simulink model "ASM_Traffic_A11"  (R2026a)
settings: Solver=ode1  StartTime=SIM.tstart.v  StopTime=SIM.tend.v  FixedStep=SIM.StepSize.v
PostLoadFcn:
  | if any(exist('dsrtsu_mdlpostloadfcn', 'file') ~= 0), dsrtsu_mdlpostloadfcn('Execute', bdroot); end
  | try, asm_mdl_postloadfcn(bdroot, 'UpdateModel', 3600); catch, disp(lasterr); end,
InitFcn:
  | , if any(exist('rtifpga_mdlclblib', 'file') ~= 0), rtifpga_mdlclblib('Init', bdroot); end,
  | , if any(exist('dsmpb_private', 'file') ~= 0), dsmpb_private('dsmpb_mdlclblib', 'Init', bdroot); end,
undefined symbols (not defined in the file): _to_, a0b2, ASM_BrakeHydraulics_DemoSystems, ASM_VehicleDynamics_DemoSystems, b98103fe8ad365046cd0, BrakeCircuit, controllerConfig, CPT, Crankshaft, DiscIntNeverNeededParam, dsmsi, FinalDriveAssembly, instance, MDL, ModeSignals, mu, Pos_BrakePedal_Maneuver, rad, RefSignals, s_to_rpm, SIM, SoftECU, Suspension, Tire, Transmission
libraries: ASM_Traffic_lib x135, simulink x98, ASM_Utils_lib x77, ASM_VehicleDynamics_lib x70, ASM_Environment_lib x22, dsmpblib x20, dsmsilib x15, MDLD_Utils_lib x10, ASM_BrakeHydraulics_lib x3, sl_discontinuities x2
(part 46 of 63)

== system ASM_Traffic_A11/Environment/GroundTruth/UserInterface/PAR_Plant/Fellow_Vehicles/Lightstates_Fellow24 ==
  Fellow_Indicator_State[] : Inport
  Brake[] : Constant  Tag=AD:ASM_Sw_SpeedLimit_Source[1Manual|2RoadScenery]  Value=2
  Emergency_Vehicle_Illumination[] : Constant  Tag=AD:ASM_Sw_SpeedLimit_Source[1Manual|2RoadScenery]  Value=2
  Front_Fog_Light[] : Constant  Tag=AD:ASM_Sw_SpeedLimit_Source[1Manual|2RoadScenery]  Value=2
  Head_Light[] : Constant  Tag=AD:ASM_Sw_SpeedLimit_Source[1Manual|2RoadScenery]  Value=2
  High_Beam[] : Constant  Tag=AD:ASM_Sw_SpeedLimit_Source[1Manual|2RoadScenery]  Value=2
  Indicator_State[] : Subsystem
  License_Plate_Illumination_Rear[] : Constant  Tag=AD:ASM_Sw_SpeedLimit_Source[1Manual|2RoadScenery]  Value=2
  Mux : Mux  Inputs=10
  Rear_Fog_Light[] : Constant  Tag=AD:ASM_Sw_SpeedLimit_Source[1Manual|2RoadScenery]  Value=2
  Reversing_Light[] : Constant  Tag=AD:ASM_Sw_SpeedLimit_Source[1Manual|2RoadScenery]  Value=2
  Service_Vehicle_Illumination[] : Constant  Tag=AD:ASM_Sw_SpeedLimit_Source[1Manual|2RoadScenery]  Value=2
  Lightstates[] : Outport  VectorParamsAs1DForOutWhenUnconnected=off
  wires:
  Service_Vehicle_Illumination[]/1 -> Mux/8
  Emergency_Vehicle_Illumination[]/1 -> Mux/7
  License_Plate_Illumination_Rear[]/1 -> Mux/5
  Front_Fog_Light[]/1 -> Mux/3
  Rear_Fog_Light[]/1 -> Mux/6
  Brake[]/1 -> Mux/10
  Head_Light[]/1 -> Mux/4
  High_Beam[]/1 -> Mux/1
  Reversing_Light[]/1 -> Mux/2
  Indicator_State[]/1(Indicator_State[]) -> Mux/9
  Mux/1 -> Lightstates[]/1  "LightStates[]"
  Fellow_Indicator_State[]/1 -> Indicator_State[]/1(Fellow_TurnLights[])

== system ASM_Traffic_A11/Environment/GroundTruth/UserInterface/PAR_Plant/Fellow_Vehicles/Lightstates_Fellow25 ==
  Fellow_Indicator_State[] : Inport
  Brake[] : Constant  Tag=AD:ASM_Sw_SpeedLimit_Source[1Manual|2RoadScenery]  Value=2
  Emergency_Vehicle_Illumination[] : Constant  Tag=AD:ASM_Sw_SpeedLimit_Source[1Manual|2RoadScenery]  Value=2
  Front_Fog_Light[] : Constant  Tag=AD:ASM_Sw_SpeedLimit_Source[1Manual|2RoadScenery]  Value=2
  Head_Light[] : Constant  Tag=AD:ASM_Sw_SpeedLimit_Source[1Manual|2RoadScenery]  Value=2
  High_Beam[] : Constant  Tag=AD:ASM_Sw_SpeedLimit_Source[1Manual|2RoadScenery]  Value=2
  Indicator_State[] : Subsystem
  License_Plate_Illumination_Rear[] : Constant  Tag=AD:ASM_Sw_SpeedLimit_Source[1Manual|2RoadScenery]  Value=2
  Mux : Mux  Inputs=10
  Rear_Fog_Light[] : Constant  Tag=AD:ASM_Sw_SpeedLimit_Source[1Manual|2RoadScenery]  Value=2
  Reversing_Light[] : Constant  Tag=AD:ASM_Sw_SpeedLimit_Source[1Manual|2RoadScenery]  Value=2
  Service_Vehicle_Illumination[] : Constant  Tag=AD:ASM_Sw_SpeedLimit_Source[1Manual|2RoadScenery]  Value=2
  Lightstates[] : Outport  VectorParamsAs1DForOutWhenUnconnected=off
  wires:
  Fellow_Indicator_State[]/1 -> Indicator_State[]/1(Fellow_TurnLights[])
  Mux/1 -> Lightstates[]/1  "LightStates[]"
  Indicator_State[]/1(Indicator_State[]) -> Mux/9
  Reversing_Light[]/1 -> Mux/2
  High_Beam[]/1 -> Mux/1
  Head_Light[]/1 -> Mux/4
  Brake[]/1 -> Mux/10
  Rear_Fog_Light[]/1 -> Mux/6
  Front_Fog_Light[]/1 -> Mux/3
  License_Plate_Illumination_Rear[]/1 -> Mux/5
  Emergency_Vehicle_Illumination[]/1 -> Mux/7
  Service_Vehicle_Illumination[]/1 -> Mux/8

== system ASM_Traffic_A11/Environment/GroundTruth/UserInterface/PAR_Plant/Fellow_Vehicles/Lightstates_Fellow26 ==
  Fellow_Indicator_State[] : Inport
  Brake[] : Constant  Tag=AD:ASM_Sw_SpeedLimit_Source[1Manual|2RoadScenery]  Value=2
  Emergency_Vehicle_Illumination[] : Constant  Tag=AD:ASM_Sw_SpeedLimit_Source[1Manual|2RoadScenery]  Value=2
  Front_Fog_Light[] : Constant  Tag=AD:ASM_Sw_SpeedLimit_Source[1Manual|2RoadScenery]  Value=2
  Head_Light[] : Constant  Tag=AD:ASM_Sw_SpeedLimit_Source[1Manual|2RoadScenery]  Value=2
  High_Beam[] : Constant  Tag=AD:ASM_Sw_SpeedLimit_Source[1Manual|2RoadScenery]  Value=2
  Indicator_State[] : Subsystem
  License_Plate_Illumination_Rear[] : Constant  Tag=AD:ASM_Sw_SpeedLimit_Source[1Manual|2RoadScenery]  Value=2
  Mux : Mux  Inputs=10
  Rear_Fog_Light[] : Constant  Tag=AD:ASM_Sw_SpeedLimit_Source[1Manual|2RoadScenery]  Value=2
  Reversing_Light[] : Constant  Tag=AD:ASM_Sw_SpeedLimit_Source[1Manual|2RoadScenery]  Value=2
  Service_Vehicle_Illumination[] : Constant  Tag=AD:ASM_Sw_SpeedLimit_Source[1Manual|2RoadScenery]  Value=2
  Lightstates[] : Outport  VectorParamsAs1DForOutWhenUnconnected=off
  wires:
  Service_Vehicle_Illumination[]/1 -> Mux/8
  Emergency_Vehicle_Illumination[]/1 -> Mux/7
  License_Plate_Illumination_Rear[]/1 -> Mux/5
  Front_Fog_Light[]/1 -> Mux/3
  Rear_Fog_Light[]/1 -> Mux/6
  Brake[]/1 -> Mux/10
  Head_Light[]/1 -> Mux/4
  High_Beam[]/1 -> Mux/1
  Reversing_Light[]/1 -> Mux/2
  Indicator_State[]/1(Indicator_State[]) -> Mux/9
  Mux/1 -> Lightstates[]/1  "LightStates[]"
  Fellow_Indicator_State[]/1 -> Indicator_State[]/1(Fellow_TurnLights[])

== system ASM_Traffic_A11/Environment/GroundTruth/UserInterface/PAR_Plant/Fellow_Vehicles/Lightstates_Fellow27 ==
  Fellow_Indicator_State[] : Inport
  Brake[] : Constant  Tag=AD:ASM_Sw_SpeedLimit_Source[1Manual|2RoadScenery]  Value=2
  Emergency_Vehicle_Illumination[] : Constant  Tag=AD:ASM_Sw_SpeedLimit_Source[1Manual|2RoadScenery]  Value=2
  Front_Fog_Light[] : Constant  Tag=AD:ASM_Sw_SpeedLimit_Source[1Manual|2RoadScenery]  Value=2
  Head_Light[] : Constant  Tag=AD:ASM_Sw_SpeedLimit_Source[1Manual|2RoadScenery]  Value=2
  High_Beam[] : Constant  Tag=AD:ASM_Sw_SpeedLimit_Source[1Manual|2RoadScenery]  Value=2
  Indicator_State[] : Subsystem
  License_Plate_Illumination_Rear[] : Constant  Tag=AD:ASM_Sw_SpeedLimit_Source[1Manual|2RoadScenery]  Value=2
  Mux : Mux  Inputs=10
  Rear_Fog_Light[] : Constant  Tag=AD:ASM_Sw_SpeedLimit_Source[1Manual|2RoadScenery]  Value=2
  Reversing_Light[] : Constant  Tag=AD:ASM_Sw_SpeedLimit_Source[1Manual|2RoadScenery]  Value=2
  Service_Vehicle_Illumination[] : Constant  Tag=AD:ASM_Sw_SpeedLimit_Source[1Manual|2RoadScenery]  Value=2
  Lightstates[] : Outport  VectorParamsAs1DForOutWhenUnconnected=off
  wires:
  Fellow_Indicator_State[]/1 -> Indicator_State[]/1(Fellow_TurnLights[])
  Mux/1 -> Lightstates[]/1  "LightStates[]"
  Indicator_State[]/1(Indicator_State[]) -> Mux/9
  Reversing_Light[]/1 -> Mux/2
  High_Beam[]/1 -> Mux/1
  Head_Light[]/1 -> Mux/4
  Brake[]/1 -> Mux/10
  Rear_Fog_Light[]/1 -> Mux/6
  Front_Fog_Light[]/1 -> Mux/3
  License_Plate_Illumination_Rear[]/1 -> Mux/5
  Emergency_Vehicle_Illumination[]/1 -> Mux/7
  Service_Vehicle_Illumination[]/1 -> Mux/8

== system ASM_Traffic_A11/Environment/GroundTruth/UserInterface/PAR_Plant/Fellow_Vehicles/Lightstates_Fellow28 ==
  Fellow_Indicator_State[] : Inport
  Brake[] : Constant  Tag=AD:ASM_Sw_SpeedLimit_Source[1Manual|2RoadScenery]  Value=2
  Emergency_Vehicle_Illumination[] : Constant  Tag=AD:ASM_Sw_SpeedLimit_Source[1Manual|2RoadScenery]  Value=2
  Front_Fog_Light[] : Constant  Tag=AD:ASM_Sw_SpeedLimit_Source[1Manual|2RoadScenery]  Value=2
  Head_Light[] : Constant  Tag=AD:ASM_Sw_SpeedLimit_Source[1Manual|2RoadScenery]  Value=2
  High_Beam[] : Constant  Tag=AD:ASM_Sw_SpeedLimit_Source[1Manual|2RoadScenery]  Value=2
  Indicator_State[] : Subsystem
  License_Plate_Illumination_Rear[] : Constant  Tag=AD:ASM_Sw_SpeedLimit_Source[1Manual|2RoadScenery]  Value=2
  Mux : Mux  Inputs=10
  Rear_Fog_Light[] : Constant  Tag=AD:ASM_Sw_SpeedLimit_Source[1Manual|2RoadScenery]  Value=2
  Reversing_Light[] : Constant  Tag=AD:ASM_Sw_SpeedLimit_Source[1Manual|2RoadScenery]  Value=2
  Service_Vehicle_Illumination[] : Constant  Tag=AD:ASM_Sw_SpeedLimit_Source[1Manual|2RoadScenery]  Value=2
  Lightstates[] : Outport  VectorParamsAs1DForOutWhenUnconnected=off
  wires:
  Service_Vehicle_Illumination[]/1 -> Mux/8
  Emergency_Vehicle_Illumination[]/1 -> Mux/7
  License_Plate_Illumination_Rear[]/1 -> Mux/5
  Front_Fog_Light[]/1 -> Mux/3
  Rear_Fog_Light[]/1 -> Mux/6
  Brake[]/1 -> Mux/10
  Head_Light[]/1 -> Mux/4
  High_Beam[]/1 -> Mux/1
  Reversing_Light[]/1 -> Mux/2
  Indicator_State[]/1(Indicator_State[]) -> Mux/9
  Mux/1 -> Lightstates[]/1  "LightStates[]"
  Fellow_Indicator_State[]/1 -> Indicator_State[]/1(Fellow_TurnLights[])

== system ASM_Traffic_A11/Environment/GroundTruth/UserInterface/PAR_Plant/Fellow_Vehicles/Lightstates_Fellow29 ==
  Fellow_Indicator_State[] : Inport
  Brake[] : Constant  Tag=AD:ASM_Sw_SpeedLimit_Source[1Manual|2RoadScenery]  Value=2
  Emergency_Vehicle_Illumination[] : Constant  Tag=AD:ASM_Sw_SpeedLimit_Source[1Manual|2RoadScenery]  Value=2
  Front_Fog_Light[] : Constant  Tag=AD:ASM_Sw_SpeedLimit_Source[1Manual|2RoadScenery]  Value=2
  Head_Light[] : Constant  Tag=AD:ASM_Sw_SpeedLimit_Source[1Manual|2RoadScenery]  Value=2
  High_Beam[] : Constant  Tag=AD:ASM_Sw_SpeedLimit_Source[1Manual|2RoadScenery]  Value=2
  Indicator_State[] : Subsystem
  License_Plate_Illumination_Rear[] : Constant  Tag=AD:ASM_Sw_SpeedLimit_Source[1Manual|2RoadScenery]  Value=2
  Mux : Mux  Inputs=10
  Rear_Fog_Light[] : Constant  Tag=AD:ASM_Sw_SpeedLimit_Source[1Manual|2RoadScenery]  Value=2
  Reversing_Light[] : Constant  Tag=AD:ASM_Sw_SpeedLimit_Source[1Manual|2RoadScenery]  Value=2
  Service_Vehicle_Illumination[] : Constant  Tag=AD:ASM_Sw_SpeedLimit_Source[1Manual|2RoadScenery]  Value=2
  Lightstates[] : Outport  VectorParamsAs1DForOutWhenUnconnected=off
  wires:
  Fellow_Indicator_State[]/1 -> Indicator_State[]/1(Fellow_TurnLights[])
  Mux/1 -> Lightstates[]/1  "LightStates[]"
  Indicator_State[]/1(Indicator_State[]) -> Mux/9
  Reversing_Light[]/1 -> Mux/2
  High_Beam[]/1 -> Mux/1
  Head_Light[]/1 -> Mux/4
  Brake[]/1 -> Mux/10
  Rear_Fog_Light[]/1 -> Mux/6
  Front_Fog_Light[]/1 -> Mux/3
  License_Plate_Illumination_Rear[]/1 -> Mux/5
  Emergency_Vehicle_Illumination[]/1 -> Mux/7
  Service_Vehicle_Illumination[]/1 -> Mux/8

== system ASM_Traffic_A11/Environment/GroundTruth/UserInterface/PAR_Plant/Fellow_Vehicles/Lightstates_Fellow3 ==
  Fellow_Indicator_State[] : Inport
  Brake[] : Constant  Tag=AD:ASM_Sw_SpeedLimit_Source[1Manual|2RoadScenery]  Value=2
  Emergency_Vehicle_Illumination[] : Constant  Tag=AD:ASM_Sw_SpeedLimit_Source[1Manual|2RoadScenery]  Value=2
  Front_Fog_Light[] : Constant  Tag=AD:ASM_Sw_SpeedLimit_Source[1Manual|2RoadScenery]  Value=2
  Head_Light[] : Constant  Tag=AD:ASM_Sw_SpeedLimit_Source[1Manual|2RoadScenery]  Value=2
  High_Beam[] : Constant  Tag=AD:ASM_Sw_SpeedLimit_Source[1Manual|2RoadScenery]  Value=2
  Indicator_State[] : Subsystem
  License_Plate_Illumination_Rear[] : Constant  Tag=AD:ASM_Sw_SpeedLimit_Source[1Manual|2RoadScenery]  Value=2
  Mux : Mux  Inputs=10
  Rear_Fog_Light[] : Constant  Tag=AD:ASM_Sw_SpeedLimit_Source[1Manual|2RoadScenery]  Value=2
  Reversing_Light[] : Constant  Tag=AD:ASM_Sw_SpeedLimit_Source[1Manual|2RoadScenery]  Value=2
  Service_Vehicle_Illumination[] : Constant  Tag=AD:ASM_Sw_SpeedLimit_Source[1Manual|2RoadScenery]  Value=2
  Lightstates[] : Outport  VectorParamsAs1DForOutWhenUnconnected=off
  wires:
  Fellow_Indicator_State[]/1 -> Indicator_State[]/1(Fellow_TurnLights[])
  Mux/1 -> Lightstates[]/1  "LightStates[]"
  Indicator_State[]/1(Indicator_State[]) -> Mux/9
  Reversing_Light[]/1 -> Mux/2
  High_Beam[]/1 -> Mux/1
  Head_Light[]/1 -> Mux/4
  Brake[]/1 -> Mux/10
  Rear_Fog_Light[]/1 -> Mux/6
  Front_Fog_Light[]/1 -> Mux/3
  License_Plate_Illumination_Rear[]/1 -> Mux/5
  Emergency_Vehicle_Illumination[]/1 -> Mux/7
  Service_Vehicle_Illumination[]/1 -> Mux/8

== system ASM_Traffic_A11/Environment/GroundTruth/UserInterface/PAR_Plant/Fellow_Vehicles/Lightstates_Fellow30 ==
  Fellow_Indicator_State[] : Inport
  Brake[] : Constant  Tag=AD:ASM_Sw_SpeedLimit_Source[1Manual|2RoadScenery]  Value=2
  Emergency_Vehicle_Illumination[] : Constant  Tag=AD:ASM_Sw_SpeedLimit_Source[1Manual|2RoadScenery]  Value=2
  Front_Fog_Light[] : Constant  Tag=AD:ASM_Sw_SpeedLimit_Source[1Manual|2RoadScenery]  Value=2
  Head_Light[] : Constant  Tag=AD:ASM_Sw_SpeedLimit_Source[1Manual|2RoadScenery]  Value=2
  High_Beam[] : Constant  Tag=AD:ASM_Sw_SpeedLimit_Source[1Manual|2RoadScenery]  Value=2
  Indicator_State[] : Subsystem
  License_Plate_Illumination_Rear[] : Constant  Tag=AD:ASM_Sw_SpeedLimit_Source[1Manual|2RoadScenery]  Value=2
  Mux : Mux  Inputs=10
  Rear_Fog_Light[] : Constant  Tag=AD:ASM_Sw_SpeedLimit_Source[1Manual|2RoadScenery]  Value=2
  Reversing_Light[] : Constant  Tag=AD:ASM_Sw_SpeedLimit_Source[1Manual|2RoadScenery]  Value=2
  Service_Vehicle_Illumination[] : Constant  Tag=AD:ASM_Sw_SpeedLimit_Source[1Manual|2RoadScenery]  Value=2
  Lightstates[] : Outport  VectorParamsAs1DForOutWhenUnconnected=off
  wires:
  Service_Vehicle_Illumination[]/1 -> Mux/8
  Emergency_Vehicle_Illumination[]/1 -> Mux/7
  License_Plate_Illumination_Rear[]/1 -> Mux/5
  Front_Fog_Light[]/1 -> Mux/3
  Rear_Fog_Light[]/1 -> Mux/6
  Brake[]/1 -> Mux/10
  Head_Light[]/1 -> Mux/4
  High_Beam[]/1 -> Mux/1
  Reversing_Light[]/1 -> Mux/2
  Indicator_State[]/1(Indicator_State[]) -> Mux/9
  Mux/1 -> Lightstates[]/1  "LightStates[]"
  Fellow_Indicator_State[]/1 -> Indicator_State[]/1(Fellow_TurnLights[])

== system ASM_Traffic_A11/Environment/GroundTruth/UserInterface/PAR_Plant/Fellow_Vehicles/Lightstates_Fellow4 ==
  Fellow_Indicator_State[] : Inport
  Brake[] : Constant  Tag=AD:ASM_Sw_SpeedLimit_Source[1Manual|2RoadScenery]  Value=2
  Emergency_Vehicle_Illumination[] : Constant  Tag=AD:ASM_Sw_SpeedLimit_Source[1Manual|2RoadScenery]  Value=2
  Front_Fog_Light[] : Constant  Tag=AD:ASM_Sw_SpeedLimit_Source[1Manual|2RoadScenery]  Value=2
  Head_Light[] : Constant  Tag=AD:ASM_Sw_SpeedLimit_Source[1Manual|2RoadScenery]  Value=2
  High_Beam[] : Constant  Tag=AD:ASM_Sw_SpeedLimit_Source[1Manual|2RoadScenery]  Value=2
  Indicator_State[] : Subsystem
  License_Plate_Illumination_Rear[] : Constant  Tag=AD:ASM_Sw_SpeedLimit_Source[1Manual|2RoadScenery]  Value=2
  Mux : Mux  Inputs=10
  Rear_Fog_Light[] : Constant  Tag=AD:ASM_Sw_SpeedLimit_Source[1Manual|2RoadScenery]  Value=2
  Reversing_Light[] : Constant  Tag=AD:ASM_Sw_SpeedLimit_Source[1Manual|2RoadScenery]  Value=2
  Service_Vehicle_Illumination[] : Constant  Tag=AD:ASM_Sw_SpeedLimit_Source[1Manual|2RoadScenery]  Value=2
  Lightstates[] : Outport  VectorParamsAs1DForOutWhenUnconnected=off
  wires:
  Service_Vehicle_Illumination[]/1 -> Mux/8
  Emergency_Vehicle_Illumination[]/1 -> Mux/7
  License_Plate_Illumination_Rear[]/1 -> Mux/5
  Front_Fog_Light[]/1 -> Mux/3
  Rear_Fog_Light[]/1 -> Mux/6
  Brake[]/1 -> Mux/10
  Head_Light[]/1 -> Mux/4
  High_Beam[]/1 -> Mux/1
  Reversing_Light[]/1 -> Mux/2
  Indicator_State[]/1(Indicator_State[]) -> Mux/9
  Mux/1 -> Lightstates[]/1  "LightStates[]"
  Fellow_Indicator_State[]/1 -> Indicator_State[]/1(Fellow_TurnLights[])

== system ASM_Traffic_A11/Environment/GroundTruth/UserInterface/PAR_Plant/Fellow_Vehicles/Lightstates_Fellow5 ==
  Fellow_Indicator_State[] : Inport
  Brake[] : Constant  Tag=AD:ASM_Sw_SpeedLimit_Source[1Manual|2RoadScenery]  Value=2
  Emergency_Vehicle_Illumination[] : Constant  Tag=AD:ASM_Sw_SpeedLimit_Source[1Manual|2RoadScenery]  Value=2
  Front_Fog_Light[] : Constant  Tag=AD:ASM_Sw_SpeedLimit_Source[1Manual|2RoadScenery]  Value=2
  Head_Light[] : Constant  Tag=AD:ASM_Sw_SpeedLimit_Source[1Manual|2RoadScenery]  Value=2
  High_Beam[] : Constant  Tag=AD:ASM_Sw_SpeedLimit_Source[1Manual|2RoadScenery]  Value=2
  Indicator_State[] : Subsystem
  License_Plate_Illumination_Rear[] : Constant  Tag=AD:ASM_Sw_SpeedLimit_Source[1Manual|2RoadScenery]  Value=2
  Mux : Mux  Inputs=10
  Rear_Fog_Light[] : Constant  Tag=AD:ASM_Sw_SpeedLimit_Source[1Manual|2RoadScenery]  Value=2
  Reversing_Light[] : Constant  Tag=AD:ASM_Sw_SpeedLimit_Source[1Manual|2RoadScenery]  Value=2
  Service_Vehicle_Illumination[] : Constant  Tag=AD:ASM_Sw_SpeedLimit_Source[1Manual|2RoadScenery]  Value=2
  Lightstates[] : Outport  VectorParamsAs1DForOutWhenUnconnected=off
  wires:
  Fellow_Indicator_State[]/1 -> Indicator_State[]/1(Fellow_TurnLights[])
  Mux/1 -> Lightstates[]/1  "LightStates[]"
  Indicator_State[]/1(Indicator_State[]) -> Mux/9
  Reversing_Light[]/1 -> Mux/2
  High_Beam[]/1 -> Mux/1
  Head_Light[]/1 -> Mux/4
  Brake[]/1 -> Mux/10
  Rear_Fog_Light[]/1 -> Mux/6
  Front_Fog_Light[]/1 -> Mux/3
  License_Plate_Illumination_Rear[]/1 -> Mux/5
  Emergency_Vehicle_Illumination[]/1 -> Mux/7
  Service_Vehicle_Illumination[]/1 -> Mux/8

== system ASM_Traffic_A11/Environment/GroundTruth/UserInterface/PAR_Plant/Fellow_Vehicles/Lightstates_Fellow6 ==
  Fellow_Indicator_State[] : Inport
  Brake[] : Constant  Tag=AD:ASM_Sw_SpeedLimit_Source[1Manual|2RoadScenery]  Value=2
  Emergency_Vehicle_Illumination[] : Constant  Tag=AD:ASM_Sw_SpeedLimit_Source[1Manual|2RoadScenery]  Value=2
  Front_Fog_Light[] : Constant  Tag=AD:ASM_Sw_SpeedLimit_Source[1Manual|2RoadScenery]  Value=2
  Head_Light[] : Constant  Tag=AD:ASM_Sw_SpeedLimit_Source[1Manual|2RoadScenery]  Value=2
  High_Beam[] : Constant  Tag=AD:ASM_Sw_SpeedLimit_Source[1Manual|2RoadScenery]  Value=2
  Indicator_State[] : Subsystem
  License_Plate_Illumination_Rear[] : Constant  Tag=AD:ASM_Sw_SpeedLimit_Source[1Manual|2RoadScenery]  Value=2
  Mux : Mux  Inputs=10
  Rear_Fog_Light[] : Constant  Tag=AD:ASM_Sw_SpeedLimit_Source[1Manual|2RoadScenery]  Value=2
  Reversing_Light[] : Constant  Tag=AD:ASM_Sw_SpeedLimit_Source[1Manual|2RoadScenery]  Value=2
  Service_Vehicle_Illumination[] : Constant  Tag=AD:ASM_Sw_SpeedLimit_Source[1Manual|2RoadScenery]  Value=2
  Lightstates[] : Outport  VectorParamsAs1DForOutWhenUnconnected=off
  wires:
  Service_Vehicle_Illumination[]/1 -> Mux/8
  Emergency_Vehicle_Illumination[]/1 -> Mux/7
  License_Plate_Illumination_Rear[]/1 -> Mux/5
  Front_Fog_Light[]/1 -> Mux/3
  Rear_Fog_Light[]/1 -> Mux/6
  Brake[]/1 -> Mux/10
  Head_Light[]/1 -> Mux/4
  High_Beam[]/1 -> Mux/1
  Reversing_Light[]/1 -> Mux/2
  Indicator_State[]/1(Indicator_State[]) -> Mux/9
  Mux/1 -> Lightstates[]/1  "LightStates[]"
  Fellow_Indicator_State[]/1 -> Indicator_State[]/1(Fellow_TurnLights[])

== system ASM_Traffic_A11/Environment/GroundTruth/UserInterface/PAR_Plant/Fellow_Vehicles/Lightstates_Fellow7 ==
  Fellow_Indicator_State[] : Inport
  Brake[] : Constant  Tag=AD:ASM_Sw_SpeedLimit_Source[1Manual|2RoadScenery]  Value=2
  Emergency_Vehicle_Illumination[] : Constant  Tag=AD:ASM_Sw_SpeedLimit_Source[1Manual|2RoadScenery]  Value=2
  Front_Fog_Light[] : Constant  Tag=AD:ASM_Sw_SpeedLimit_Source[1Manual|2RoadScenery]  Value=2
  Head_Light[] : Constant  Tag=AD:ASM_Sw_SpeedLimit_Source[1Manual|2RoadScenery]  Value=2
  High_Beam[] : Constant  Tag=AD:ASM_Sw_SpeedLimit_Source[1Manual|2RoadScenery]  Value=2
  Indicator_State[] : Subsystem
  License_Plate_Illumination_Rear[] : Constant  Tag=AD:ASM_Sw_SpeedLimit_Source[1Manual|2RoadScenery]  Value=2
  Mux : Mux  Inputs=10
  Rear_Fog_Light[] : Constant  Tag=AD:ASM_Sw_SpeedLimit_Source[1Manual|2RoadScenery]  Value=2
  Reversing_Light[] : Constant  Tag=AD:ASM_Sw_SpeedLimit_Source[1Manual|2RoadScenery]  Value=2
  Service_Vehicle_Illumination[] : Constant  Tag=AD:ASM_Sw_SpeedLimit_Source[1Manual|2RoadScenery]  Value=2
  Lightstates[] : Outport  VectorParamsAs1DForOutWhenUnconnected=off
  wires:
  Fellow_Indicator_State[]/1 -> Indicator_State[]/1(Fellow_TurnLights[])
  Mux/1 -> Lightstates[]/1  "LightStates[]"
  Indicator_State[]/1(Indicator_State[]) -> Mux/9
  Reversing_Light[]/1 -> Mux/2
  High_Beam[]/1 -> Mux/1
  Head_Light[]/1 -> Mux/4
  Brake[]/1 -> Mux/10
  Rear_Fog_Light[]/1 -> Mux/6
  Front_Fog_Light[]/1 -> Mux/3
  License_Plate_Illumination_Rear[]/1 -> Mux/5
  Emergency_Vehicle_Illumination[]/1 -> Mux/7
  Service_Vehicle_Illumination[]/1 -> Mux/8

== system ASM_Traffic_A11/Environment/GroundTruth/UserInterface/PAR_Plant/Fellow_Vehicles/Lightstates_Fellow8 ==
  Fellow_Indicator_State[] : Inport
  Brake[] : Constant  Tag=AD:ASM_Sw_SpeedLimit_Source[1Manual|2RoadScenery]  Value=2
  Emergency_Vehicle_Illumination[] : Constant  Tag=AD:ASM_Sw_SpeedLimit_Source[1Manual|2RoadScenery]  Value=2
  Front_Fog_Light[] : Constant  Tag=AD:ASM_Sw_SpeedLimit_Source[1Manual|2RoadScenery]  Value=2
  Head_Light[] : Constant  Tag=AD:ASM_Sw_SpeedLimit_Source[1Manual|2RoadScenery]  Value=2
  High_Beam[] : Constant  Tag=AD:ASM_Sw_SpeedLimit_Source[1Manual|2RoadScenery]  Value=2
  Indicator_State[] : Subsystem
  License_Plate_Illumination_Rear[] : Constant  Tag=AD:ASM_Sw_SpeedLimit_Source[1Manual|2RoadScenery]  Value=2
  Mux : Mux  Inputs=10
  Rear_Fog_Light[] : Constant  Tag=AD:ASM_Sw_SpeedLimit_Source[1Manual|2RoadScenery]  Value=2
  Reversing_Light[] : Constant  Tag=AD:ASM_Sw_SpeedLimit_Source[1Manual|2RoadScenery]  Value=2
  Service_Vehicle_Illumination[] : Constant  Tag=AD:ASM_Sw_SpeedLimit_Source[1Manual|2RoadScenery]  Value=2
  Lightstates[] : Outport  VectorParamsAs1DForOutWhenUnconnected=off
  wires:
  Service_Vehicle_Illumination[]/1 -> Mux/8
  Emergency_Vehicle_Illumination[]/1 -> Mux/7
  License_Plate_Illumination_Rear[]/1 -> Mux/5
  Front_Fog_Light[]/1 -> Mux/3
  Rear_Fog_Light[]/1 -> Mux/6
  Brake[]/1 -> Mux/10
  Head_Light[]/1 -> Mux/4
  High_Beam[]/1 -> Mux/1
  Reversing_Light[]/1 -> Mux/2
  Indicator_State[]/1(Indicator_State[]) -> Mux/9
  Mux/1 -> Lightstates[]/1  "LightStates[]"
  Fellow_Indicator_State[]/1 -> Indicator_State[]/1(Fellow_TurnLights[])

== system ASM_Traffic_A11/Environment/GroundTruth/UserInterface/PAR_Plant/Fellow_Vehicles/Lightstates_Fellow9 ==
  Fellow_Indicator_State[] : Inport
  Brake[] : Constant  Tag=AD:ASM_Sw_SpeedLimit_Source[1Manual|2RoadScenery]  Value=2
  Emergency_Vehicle_Illumination[] : Constant  Tag=AD:ASM_Sw_SpeedLimit_Source[1Manual|2RoadScenery]  Value=2
  Front_Fog_Light[] : Constant  Tag=AD:ASM_Sw_SpeedLimit_Source[1Manual|2RoadScenery]  Value=2
  Head_Light[] : Constant  Tag=AD:ASM_Sw_SpeedLimit_Source[1Manual|2RoadScenery]  Value=2
  High_Beam[] : Constant  Tag=AD:ASM_Sw_SpeedLimit_Source[1Manual|2RoadScenery]  Value=2
  Indicator_State[] : Subsystem
  License_Plate_Illumination_Rear[] : Constant  Tag=AD:ASM_Sw_SpeedLimit_Source[1Manual|2RoadScenery]  Value=2
  Mux : Mux  Inputs=10
  Rear_Fog_Light[] : Constant  Tag=AD:ASM_Sw_SpeedLimit_Source[1Manual|2RoadScenery]  Value=2
  Reversing_Light[] : Constant  Tag=AD:ASM_Sw_SpeedLimit_Source[1Manual|2RoadScenery]  Value=2
  Service_Vehicle_Illumination[] : Constant  Tag=AD:ASM_Sw_SpeedLimit_Source[1Manual|2RoadScenery]  Value=2
  Lightstates[] : Outport  VectorParamsAs1DForOutWhenUnconnected=off
  wires:
  Fellow_Indicator_State[]/1 -> Indicator_State[]/1(Fellow_TurnLights[])
  Mux/1 -> Lightstates[]/1  "LightStates[]"
  Indicator_State[]/1(Indicator_State[]) -> Mux/9
  Reversing_Light[]/1 -> Mux/2
  High_Beam[]/1 -> Mux/1
  Head_Light[]/1 -> Mux/4
  Brake[]/1 -> Mux/10
  Rear_Fog_Light[]/1 -> Mux/6
  Front_Fog_Light[]/1 -> Mux/3
  License_Plate_Illumination_Rear[]/1 -> Mux/5
  Emergency_Vehicle_Illumination[]/1 -> Mux/7
  Service_Vehicle_Illumination[]/1 -> Mux/8

== system ASM_Traffic_A11/Environment/GroundTruth/UserInterface/PAR_Plant/HostVehicle_Data_AutomatedDrivingFunction/AutomatedDrivingFunction_1 ==
  Interface_In : Inport
  Bus Creator : BusCreator  Inputs=10
  Bus Selector1 : BusSelector  OutputSignals=Interface_In.ExternalModel.Driver_Override_ACC_Active[0Off|1On],Interface_In.ExternalModel.Driver_Override_ACC_Reason[0NoOverride|1BrakePedal|2AccPedal],Interface_In.ExternalModel.ACC_State[1OFF|2Standby|3ON]
  Custom_Name_Idx[] : Constant  Value=0
  Custom_State_Idx[] : Constant  Value=0
  Key_1_Idx[] : Constant  Value=0
  Key_2_Idx[] : Constant  Value=0
  Mappings : Subsystem
  Name_Idx[] : Constant  Value=10
  Value_1_Idx[] : Constant  Value=0
  Value_2_Idx[] : Constant  Value=0
  AutomatedDrivingFunction_ACC[] : Outport  VectorParamsAs1DForOutWhenUnconnected=off
  wires:
  Bus Selector1/3 -> Mappings/3(ACC_State[1OFF|2Standby|3ON])  "<ACC_State[1OFF|2Standby|3ON]>"
  Interface_In/1 -> Bus Selector1/1
  Custom_Name_Idx[]/1 -> Bus Creator/5  "Custom_Name_Idx[]"
  Name_Idx[]/1 -> Bus Creator/4  "Name_Idx[]"
  Mappings/2(DriverOverride_Reason_Idx[]) -> Bus Creator/2  "Driver_Override_Reason_Idx[]"
  Bus Creator/1 -> AutomatedDrivingFunction_ACC[]/1
  Custom_State_Idx[]/1 -> Bus Creator/6  "Custom_State_Idx[]"
  Bus Selector1/1 -> Mappings/1(Driver_Override_ACC_Active_In[0Off|1On])  "<Driver_Override_ACC_Active[0Off|1On]>"
  Bus Selector1/2 -> Mappings/2(Driver_Override_ACC_Reason[0NoOverride|1BrakePedal|2AccPedal])  "<Driver_Override_ACC_Reason[0NoOverride|1BrakePedal|2AccPedal]>"
  Mappings/3(State_Idx[]) -> Bus Creator/3  "State_Idx[]"
  Key_1_Idx[]/1 -> Bus Creator/7  "Key_1_Idx[]"
  Value_1_Idx[]/1 -> Bus Creator/8  "Value_1_Idx[]"
  Key_2_Idx[]/1 -> Bus Creator/9  "Key_2_Idx[]"
  Value_2_Idx[]/1 -> Bus Creator/10  "Value_2_Idx[]"
  Mappings/1(Driver_Override_ACC_Active[0Off|1On]) -> Bus Creator/1  "Driver_Override_Active[0Off|1On]"

== system ASM_Traffic_A11/Environment/GroundTruth/UserInterface/PAR_Plant/HostVehicle_Data_AutomatedDrivingFunction/AutomatedDrivingFunction_2 ==
  Interface_In : Inport
  Bus Creator : BusCreator  Inputs=10
  Bus Selector1 : BusSelector  OutputSignals=Interface_In.ExternalModel.Driver_Override_ACC_Active[0Off|1On],Interface_In.ExternalModel.Driver_Override_ACC_Reason[0NoOverride|1BrakePedal|2AccPedal],Interface_In.ExternalModel.AEB[0|1]
  Custom_Name_Idx[] : Constant  Value=0
  Custom_State_Idx[] : Constant  Value=0
  Key_1_Idx[] : Constant  Value=0
  Key_2_Idx[] : Constant  Value=0
  Mappings : Subsystem
  Name_Idx[] : Constant  Value=7
  Value_1_Idx[] : Constant  Value=0
  Value_2_Idx[] : Constant  Value=0
  AutomatedDrivingFunction_AEB[] : Outport  VectorParamsAs1DForOutWhenUnconnected=off
  wires:
  Custom_Name_Idx[]/1 -> Bus Creator/5  "Custom_Name_Idx[]"
  Name_Idx[]/1 -> Bus Creator/4  "Name_Idx[]"
  Custom_State_Idx[]/1 -> Bus Creator/6  "Custom_State_Idx[]"
  Bus Creator/1 -> AutomatedDrivingFunction_AEB[]/1
  Interface_In/1 -> Bus Selector1/1
  Bus Selector1/2 -> Mappings/2(Driver_Override_ACC_Reason[0NoOverride|1BrakePedal|2AccPedal])  "<Driver_Override_ACC_Reason[0NoOverride|1BrakePedal|2AccPedal]>"
  Bus Selector1/3 -> Mappings/3(AEB[0|1])  "<AEB[0|1]>"
  Value_2_Idx[]/1 -> Bus Creator/10  "Value_2_Idx[]"
  Key_2_Idx[]/1 -> Bus Creator/9  "Key_2_Idx[]"
  Value_1_Idx[]/1 -> Bus Creator/8  "Value_1_Idx[]"
  Key_1_Idx[]/1 -> Bus Creator/7  "Key_1_Idx[]"
  Bus Selector1/1 -> Mappings/1(Driver_Override_ACC_Active_In[0Off|1On])  "<Driver_Override_ACC_Active[0Off|1On]>"
  Mappings/1(Driver_Override_ACC_Active[0Off|1On]) -> Bus Creator/1  "Driver_Override_Active[0Off|1On]"
  Mappings/2(DriverOverride_Reason_Idx[]) -> Bus Creator/2  "Driver_Override_Reason_Idx[]"
  Mappings/3(State_Idx[]) -> Bus Creator/3  "State_Idx[]"

== system ASM_Traffic_A11/Environment/GroundTruth/UserInterface/PAR_Plant/HostVehicle_Data_AutomatedDrivingFunction/AutomatedDrivingFunction_3 ==
  Interface_In : Inport
  Bus Creator : BusCreator  Inputs=10
  Bus Selector1 : BusSelector  OutputSignals=Interface_In.ExternalModel.Driver_Override_ACC_Active[0Off|1On],Interface_In.ExternalModel.Driver_Override_ACC_Reason[0NoOverride|1BrakePedal|2AccPedal],Interface_In.ExternalModel.FCW[0|1]
  Custom_Name_Idx[] : Constant  Value=0
  Custom_State_Idx[] : Constant  Value=0
  Key_1_Idx[] : Constant  Value=0
  Key_2_Idx[] : Constant  Value=0
  Mappings : Subsystem
  Name_Idx[] : Constant  Value=3
  Value_1_Idx[] : Constant  Value=0
  Value_2_Idx[] : Constant  Value=0
  AutomatedDrivingFunction_FCW[] : Outport  VectorParamsAs1DForOutWhenUnconnected=off
  wires:
  Custom_Name_Idx[]/1 -> Bus Creator/5  "Custom_Name_Idx[]"
  Name_Idx[]/1 -> Bus Creator/4  "Name_Idx[]"
  Custom_State_Idx[]/1 -> Bus Creator/6  "Custom_State_Idx[]"
  Bus Creator/1 -> AutomatedDrivingFunction_FCW[]/1
  Bus Selector1/3 -> Mappings/3(FCW[0|1])  "<FCW[0|1]>"
  Interface_In/1 -> Bus Selector1/1
  Bus Selector1/2 -> Mappings/2(Driver_Override_ACC_Reason[0NoOverride|1BrakePedal|2AccPedal])  "<Driver_Override_ACC_Reason[0NoOverride|1BrakePedal|2AccPedal]>"
  Value_2_Idx[]/1 -> Bus Creator/10  "Value_2_Idx[]"
  Key_2_Idx[]/1 -> Bus Creator/9  "Key_2_Idx[]"
  Value_1_Idx[]/1 -> Bus Creator/8  "Value_1_Idx[]"
  Key_1_Idx[]/1 -> Bus Creator/7  "Key_1_Idx[]"
  Bus Selector1/1 -> Mappings/1(Driver_Override_ACC_Active_In[0Off|1On])  "<Driver_Override_ACC_Active[0Off|1On]>"
  Mappings/1(Driver_Override_ACC_Active[0Off|1On]) -> Bus Creator/1  "Driver_Override_Active[0Off|1On]"
  Mappings/3(State_Idx[]) -> Bus Creator/3  "State_Idx[]"
  Mappings/2(DriverOverride_Reason_Idx[]) -> Bus Creator/2  "Driver_Override_Reason_Idx[]"

== system ASM_Traffic_A11/Environment/GroundTruth/UserInterface/PAR_Plant/HostVehicle_Data_AutomatedDrivingFunction/AutomatedDrivingFunction_4 ==
  Interface_In : Inport
  Bus Creator : BusCreator  Inputs=10
  Custom_Name_Idx[] : Constant  Value=0
  Custom_State_Idx[] : Constant  Value=0
  Driver_Override_Active[0Off|1On] : Constant  Value=0
  Driver_Override_Reason_Idx[] : Constant  Value=0
  Key_1_Idx[] : Constant  Value=0
  Key_2_Idx[] : Constant  Value=0
  Name_Idx[] : Constant  Value=0
  State_Idx[] : Constant  Value=0
  Terminator : Terminator
  Value_1_Idx[] : Constant  Value=0
  Value_2_Idx[] : Constant  Value=0
  AutomatedDrivingFunction_4[] : Outport  VectorParamsAs1DForOutWhenUnconnected=off
  wires:
  Driver_Override_Active[0Off|1On]/1 -> Bus Creator/1  "Driver_Override_Active[0Off|1On]"
  Driver_Override_Reason_Idx[]/1 -> Bus Creator/2  "Driver_Override_Reason_Idx[]"
  Interface_In/1 -> Terminator/1
  Custom_Name_Idx[]/1 -> Bus Creator/5  "Custom_Name_Idx[]"
  Name_Idx[]/1 -> Bus Creator/4  "Name_Idx[]"
  Custom_State_Idx[]/1 -> Bus Creator/6  "Custom_State_Idx[]"
  State_Idx[]/1 -> Bus Creator/3  "State_Idx[]"
  Bus Creator/1 -> AutomatedDrivingFunction_4[]/1
  Value_2_Idx[]/1 -> Bus Creator/10  "Value_2_Idx[]"
  Key_2_Idx[]/1 -> Bus Creator/9  "Key_2_Idx[]"
  Value_1_Idx[]/1 -> Bus Creator/8  "Value_1_Idx[]"
  Key_1_Idx[]/1 -> Bus Creator/7  "Key_1_Idx[]"

== system ASM_Traffic_A11/Environment/GroundTruth/UserInterface/PAR_Plant/TrafficLight_Counter/TrafficLight_Counter_1 ==
  Bus Creator1 : BusCreator  Inputs=4
  Ext_TrafficLight_Counter_1[] : Constant  Value=0
  Multiport Switch : MultiPortSwitch  DataPortOrder=Zero-based contiguous  Inputs=2  zeroidx=on  SaturateOnIntegerOverflow=off  InputSameDT=off
  Rounding Function : Rounding  Operator=round
  Saturation : Saturate  UpperLimit=2  LowerLimit=0
  Stim_TrafficLight_Counter_1[] : Constant  Value=0
  Sw_TrafficLight_Counter_1[0Stim|1Ext] : Constant  Value=0
  TrafficLight_Counter_1[] : Outport  VectorParamsAs1DForOutWhenUnconnected=off
  wires:
  Bus Creator1/1 -> TrafficLight_Counter_1[]/1
  Stim_TrafficLight_Counter_1[]/1 -> Bus Creator1/2, Multiport Switch/2  "Stim_TrafficLight_Counter_1[]"
  Multiport Switch/1 -> Bus Creator1/4  "TrafficLight_Counter_1[]"
  Saturation/1 -> Multiport Switch/1
  Rounding Function/1 -> Saturation/1
  Ext_TrafficLight_Counter_1[]/1 -> Multiport Switch/3, Bus Creator1/3  "Ext_TrafficLight_Counter_1[]"
  Sw_TrafficLight_Counter_1[0Stim|1Ext]/1 -> Bus Creator1/1, Rounding Function/1  "Sw_TrafficLight_Counter_1[0Stim|1Ext]"

== system ASM_Traffic_A11/Environment/GroundTruth/UserInterface/PAR_Plant/TrafficLight_Counter/TrafficLight_Counter_2 ==
  Bus Creator1 : BusCreator  Inputs=4
  Ext_TrafficLight_Counter_2[] : Constant  Value=0
  Multiport Switch : MultiPortSwitch  DataPortOrder=Zero-based contiguous  Inputs=2  zeroidx=on  SaturateOnIntegerOverflow=off  InputSameDT=off
  Rounding Function : Rounding  Operator=round
  Saturation : Saturate  UpperLimit=2  LowerLimit=0
  Stim_TrafficLight_Counter_2[] : Constant  Value=0
  Sw_TrafficLight_Counter_2[0Stim|1Ext] : Constant  Value=0
  TrafficLight_Counter_2[] : Outport  VectorParamsAs1DForOutWhenUnconnected=off
  wires:
  Sw_TrafficLight_Counter_2[0Stim|1Ext]/1 -> Rounding Function/1, Bus Creator1/1  "Sw_TrafficLight_Counter_2[0Stim|1Ext]"
  Ext_TrafficLight_Counter_2[]/1 -> Bus Creator1/3, Multiport Switch/3  "Ext_TrafficLight_Counter_2[]"
  Rounding Function/1 -> Saturation/1
  Saturation/1 -> Multiport Switch/1
  Multiport Switch/1 -> Bus Creator1/4  "TrafficLight_Counter_2[]"
  Stim_TrafficLight_Counter_2[]/1 -> Multiport Switch/2, Bus Creator1/2  "Stim_TrafficLight_Counter_2[]"
  Bus Creator1/1 -> TrafficLight_Counter_2[]/1

== system ASM_Traffic_A11/Environment/GroundTruth/UserInterface/PAR_Plant/TrafficLight_Counter/TrafficLight_Counter_3 ==
  Bus Creator1 : BusCreator  Inputs=4
  Ext_TrafficLight_Counter_3[] : Constant  Value=0
  Multiport Switch : MultiPortSwitch  DataPortOrder=Zero-based contiguous  Inputs=2  zeroidx=on  SaturateOnIntegerOverflow=off  InputSameDT=off
  Rounding Function : Rounding  Operator=round
  Saturation : Saturate  UpperLimit=2  LowerLimit=0
  Stim_TrafficLight_Counter_3[] : Constant  Value=0
  Sw_TrafficLight_Counter_3[0Stim|1Ext] : Constant  Value=0
  TrafficLight_Counter_3[] : Outport  VectorParamsAs1DForOutWhenUnconnected=off
  wires:
  Bus Creator1/1 -> TrafficLight_Counter_3[]/1
  Stim_TrafficLight_Counter_3[]/1 -> Bus Creator1/2, Multiport Switch/2  "Stim_TrafficLight_Counter_3[]"
  Multiport Switch/1 -> Bus Creator1/4  "TrafficLight_Counter_3[]"
  Saturation/1 -> Multiport Switch/1
  Rounding Function/1 -> Saturation/1
  Ext_TrafficLight_Counter_3[]/1 -> Multiport Switch/3, Bus Creator1/3  "Ext_TrafficLight_Counter_3[]"
  Sw_TrafficLight_Counter_3[0Stim|1Ext]/1 -> Bus Creator1/1, Rounding Function/1  "Sw_TrafficLight_Counter_3[0Stim|1Ext]"

== system ASM_Traffic_A11/Environment/GroundTruth/UserInterface/PAR_Plant/TrafficLight_Counter/TrafficLight_Counter_4 ==
  Bus Creator1 : BusCreator  Inputs=4
  Ext_TrafficLight_Counter_4[] : Constant  Value=0
  Multiport Switch : MultiPortSwitch  DataPortOrder=Zero-based contiguous  Inputs=2  zeroidx=on  SaturateOnIntegerOverflow=off  InputSameDT=off
  Rounding Function : Rounding  Operator=round
  Saturation : Saturate  UpperLimit=2  LowerLimit=0
  Stim_TrafficLight_Counter_4[] : Constant  Value=0
  Sw_TrafficLight_Counter_4[0Stim|1Ext] : Constant  Value=0
  TrafficLight_Counter_4[] : Outport  VectorParamsAs1DForOutWhenUnconnected=off
  wires:
  Sw_TrafficLight_Counter_4[0Stim|1Ext]/1 -> Rounding Function/1, Bus Creator1/1  "Sw_TrafficLight_Counter_4[0Stim|1Ext]"
  Ext_TrafficLight_Counter_4[]/1 -> Bus Creator1/3, Multiport Switch/3  "Ext_TrafficLight_Counter_4[]"
  Rounding Function/1 -> Saturation/1
  Saturation/1 -> Multiport Switch/1
  Multiport Switch/1 -> Bus Creator1/4  "TrafficLight_Counter_4[]"
  Stim_TrafficLight_Counter_4[]/1 -> Multiport Switch/2, Bus Creator1/2  "Stim_TrafficLight_Counter_4[]"
  Bus Creator1/1 -> TrafficLight_Counter_4[]/1

== system ASM_Traffic_A11/Environment/Maneuver/PlantModel/ExternalSegmentEnd/Dist_Front_Min/Replace_NoObjectFound1 ==
  In1 : Inport
  Far_away : Constant  Value=1000
  No_Hinderance : Constant  Value=0
  Relational Operator : RelationalOperator  Operator=<=
  Switch : Switch  Threshold=1  SaturateOnIntegerOverflow=off
  Out1 : Outport  VectorParamsAs1DForOutWhenUnconnected=off
  wires:
  No_Hinderance/1 -> Relational Operator/2
  Relational Operator/1 -> Switch/2
  Far_away/1 -> Switch/1
  In1/1 -> Relational Operator/1, Switch/3
  Switch/1 -> Out1/1

== system ASM_Traffic_A11/Environment/Maneuver/PlantModel/ExternalSegmentEnd/Dist_Rear_Min/Replace_NoObjectFound1 ==
  In1 : Inport
  Far_away : Constant  Value=1000
  No_Hinderance : Constant  Value=0
  Relational Operator : RelationalOperator  Operator=<=
  Switch : Switch  Threshold=1  SaturateOnIntegerOverflow=off
  Out1 : Outport  VectorParamsAs1DForOutWhenUnconnected=off
  wires:
  Switch/1 -> Out1/1
  In1/1 -> Switch/3, Relational Operator/1
  Far_away/1 -> Switch/1
  Relational Operator/1 -> Switch/2
  No_Hinderance/1 -> Relational Operator/2

== system ASM_Traffic_A11/Environment/Maneuver/PlantModel/ExternalSegmentEnd/SegmentEndTrigger/Fishhook ==
  RollRate_Threshold[deg|s] : Inport
  RollRate_Vehicle_CoG[deg|s] : Inport  Port=2
  Abs : Abs
  Fcn_1 : Fcn  Expr=(u[1]>=0.0)*(u[2]<0.0)
  Fcn_2 : Fcn  Expr=(u[1]>0.0)
  Memory1 : UnitDelay  SampleTime=-1
  Memory2 : UnitDelay  SampleTime=-1
  Mux : Mux  Inputs=2
  Product : Product  RndMeth=Zero
  Sum : Sum  Inputs=|-+  SaturateOnIntegerOverflow=on
  SegmentEnd_Fishhook : Outport  VectorParamsAs1DForOutWhenUnconnected=off
  wires:
  Memory1/1 -> Mux/1
  Mux/1 -> Fcn_1/1
  Sum/1 -> Memory1/1, Mux/2
  Abs/1 -> Sum/2
  RollRate_Threshold[deg|s]/1 -> Sum/1, Memory2/1
  RollRate_Vehicle_CoG[deg|s]/1 -> Abs/1
  Memory2/1 -> Fcn_2/1
  Fcn_2/1 -> Product/1
  Fcn_1/1 -> Product/2
  Product/1 -> SegmentEnd_Fishhook/1

== system ASM_Traffic_A11/Environment/Maneuver/PlantModel/ExternalSegmentEnd/SegmentEndTrigger/SaturateAndRound ==
  In : Inport
  Max : Inport  Port=2
  Const_zero : Constant  Value=0
  Data Type Conversion : DataTypeConversion  SaturateOnIntegerOverflow=off  RndMeth=Floor
  Log_and : Logic  Inputs=3  AllPortsSameDT=off  OutDataTypeStr=boolean
  Product : Product  RndMeth=Zero
  RelOp1 : RelationalOperator  Operator===  OutDataTypeStr=boolean  InputSameDT=off
  RelOp2 : RelationalOperator  Operator=<=  OutDataTypeStr=boolean  InputSameDT=off
  RelOp3 : RelationalOperator  OutDataTypeStr=boolean  InputSameDT=off
  Round : Rounding  Operator=round
  ExternalSegmentEnd_Mode[] : Outport  VectorParamsAs1DForOutWhenUnconnected=off
  wires:
  In/1 -> Product/1, RelOp2/1, RelOp3/1, RelOp1/2, Round/1
  Round/1 -> RelOp1/1
  RelOp1/1 -> Log_and/1
  Log_and/1 -> Data Type Conversion/1
  Data Type Conversion/1 -> Product/2
  Const_zero/1 -> RelOp3/2
  RelOp3/1 -> Log_and/2
  RelOp2/1 -> Log_and/3
  Product/1 -> ExternalSegmentEnd_Mode[]/1
  Max/1 -> RelOp2/2

== system ASM_Traffic_A11/Environment/Maneuver/UserInterface/PAR_Plant/ManeuverControl/Enable_ManeuverStart ==
  Sw_StartManeuverAtSimStart[0|1] : Inport
  In : Inport  Port=2
  Data Type Conversion : DataTypeConversion  SaturateOnIntegerOverflow=off  RndMeth=Floor
  Logical Operator : Logic  Operator=OR  AllPortsSameDT=off  OutDataTypeStr=boolean
  Product : Product  Inputs=3
  Step : Step  Time=0.005  SampleTime=SIM.StepSize.v
  Step1 : Step  Time=0.02  InitialValue=1  FinalValue=0  SampleTime=SIM.StepSize.v
  Out : Outport  VectorParamsAs1DForOutWhenUnconnected=off
  wires:
  Step/1 -> Product/2
  Sw_StartManeuverAtSimStart[0|1]/1 -> Product/1
  Product/1 -> Logical Operator/2
  Step1/1 -> Product/3
  Logical Operator/1 -> Data Type Conversion/1
  Data Type Conversion/1 -> Out/1
  In/1 -> Logical Operator/1

== system ASM_Traffic_A11/Environment/Maneuver/UserInterface/PAR_Plant/ManeuverSettings/Replace_BrakePedal_Brake ==
  Sw_MasterBrakeCylinder_Mode[1linear|2physical] : Inport
  Pos_BrakePedal_Brake[%]_ : Inport  Port=2
  Pos_BrakePedal_BrakeUntilStop[%]_ : Inport  Port=3
  Pos_BrakePedal_Replace[%] : Inport  Port=4
  Const_physType : Constant  Value=2
  RelOpConst_physType : RelationalOperator  Operator===  OutDataTypeStr=boolean  InputSameDT=off
  Switch : Switch  Criteria=u2 ~= 0  SaturateOnIntegerOverflow=off  InputSameDT=off
  Switch1 : Switch  Criteria=u2 ~= 0  SaturateOnIntegerOverflow=off  InputSameDT=off
  Pos_BrakePedal_Brake[%] : Outport  VectorParamsAs1DForOutWhenUnconnected=off
  Pos_BrakePedal_BrakeUntilStop[%] : Outport  Port=2  VectorParamsAs1DForOutWhenUnconnected=off
  wires:
  Switch/1 -> Pos_BrakePedal_Brake[%]/1
  Const_physType/1 -> RelOpConst_physType/2
  Sw_MasterBrakeCylinder_Mode[1linear|2physical]/1 -> RelOpConst_physType/1
  RelOpConst_physType/1 -> Switch1/2, Switch/2
  Pos_BrakePedal_Replace[%]/1 -> Switch1/1, Switch/1
  Pos_BrakePedal_Brake[%]_/1 -> Switch/3
  Switch1/1 -> Pos_BrakePedal_BrakeUntilStop[%]/1
  Pos_BrakePedal_BrakeUntilStop[%]_/1 -> Switch1/3

== system ASM_Traffic_A11/Environment/Maneuver/UserInterface/PAR_Plant/ManualControl/StarterPermanentOn_Handling ==
  In1 : Inport
      settings: AttributesFormatString=Mode_StartButtonState[1Stim|2SoftECU]
  In2 : Inport  Port=2
      settings: AttributesFormatString=State_StartButton[-1PowerOff|0Acc|1PowerOn|2StarterOn]
  In3 : Inport  Port=3
  PermanentOn : simulink/Logic and Bit Operations/Compare To Constant  relop===  const=1  OutDataTypeStr=boolean
  StarterOn : Constant  Value=2
  Stim : Constant
  Switch : Switch  Criteria=u2 ~= 0  SaturateOnIntegerOverflow=off  InputSameDT=off
  Switch1 : Switch  Criteria=u2 ~= 0  SaturateOnIntegerOverflow=off  InputSameDT=off
  Out1 : Outport  VectorParamsAs1DForOutWhenUnconnected=off
  Out2 : Outport  Port=2  VectorParamsAs1DForOutWhenUnconnected=off
  wires:
  In1/1 -> Switch/3
  In2/1 -> Switch1/3
  In3/1 -> PermanentOn/1
  PermanentOn/1 -> Switch1/2, Switch/2
  Stim/1 -> Switch/1
  Switch/1 -> Out1/1
  StarterOn/1 -> Switch1/1
  Switch1/1 -> Out2/1

== system ASM_Traffic_A11/Environment/Maneuver/UserInterface/PAR_Plant/ManualControl/TestBench_Switch ==
  In1 : Inport
      settings: AttributesFormatString=Sw_Testbench[0Off|1On]
  In2 : Inport  Port=2
      settings: AttributesFormatString=EngOpNum[]
  Constant : Constant  Value=0
  Switch : Switch  Criteria=u2 ~= 0  SaturateOnIntegerOverflow=off  InputSameDT=off
  Out1 : Outport  VectorParamsAs1DForOutWhenUnconnected=off
  wires:
  Switch/1 -> Out1/1
  In2/1 -> Switch/2
  In1/1 -> Switch/1
  Constant/1 -> Switch/3

== system ASM_Traffic_A11/Environment/Road/UserInterface/PAR_Plant/BasicRoad/Subsystem ==
  Pos_CP_CoorSys_E[:][x;y][m] : Inport
  Add : Sum
  Constant : Constant
  Demux : Demux  Outputs=2
  Gain : Gain  Gain=0
  Terminator : Terminator
  Out1 : Outport  VectorParamsAs1DForOutWhenUnconnected=off
  wires:
  Gain/1 -> Add/1
  Demux/2 -> Terminator/1
  Pos_CP_CoorSys_E[:][x;y][m]/1 -> Demux/1
  Demux/1 -> Gain/1
  Add/1 -> Out1/1
  Constant/1 -> Add/2

== system ASM_Traffic_A11/Environment/Road/UserInterface/PAR_Plant/Objects_DataStreams/DataStream_1 ==
  Maneuver_Signals[] : Inport
  Bus Creator1 : BusCreator  Inputs=4
  Bus Selector : BusSelector  OutputSignals=ManeuverState[]
  Compare To Constant : simulink/Logic and Bit Operations/Compare To Constant  relop=>=  const=3.0  OutDataTypeStr=boolean
  Multiport Switch : MultiPortSwitch  DataPortOrder=Zero-based contiguous  Inputs=2  zeroidx=on  SaturateOnIntegerOverflow=off  InputSameDT=off
  Rounding Function : Rounding  Operator=round
  Saturation : Saturate  UpperLimit=1  LowerLimit=0
  Selector : Selector  InputPortWidth=4  IndexOptions=Index vector (port)  Indices=[1 3]  OutputSizes=1
  Stim_DataStream_1[] : Constant  Value=3
  Sw_DataStream_1[0Stim|1Ext] : Constant
  TrafficLight1_Control : Subsystem
  TrafficLightState[1Red|2Yellow|3RedYellow|4Green] : Constant  Value=[1 3 4 2]  VectorParams1D=off
  DataStream_1[] : Outport  VectorParamsAs1DForOutWhenUnconnected=off
  wires:
  Compare To Constant/1 -> TrafficLight1_Control/1(Reset[])
  Bus Selector/1 -> Compare To Constant/1  "<ManeuverState[]>"
  Maneuver_Signals[]/1 -> Bus Selector/1
  TrafficLightState[1Red|2Yellow|3RedYellow|4Green]/1 -> Selector/1
  Stim_DataStream_1[]/1 -> Selector/2
  Bus Creator1/1 -> DataStream_1[]/1
  Selector/1 -> Bus Creator1/2, Multiport Switch/2  "Stim_DataStream_1[]"
  Multiport Switch/1 -> Bus Creator1/4  "DataStream_1[]"
  Saturation/1 -> Multiport Switch/1
  Rounding Function/1 -> Saturation/1
  TrafficLight1_Control/1(TrafficLightState[1|2|3|4]) -> Multiport Switch/3, Bus Creator1/3  "Ext_DataStream_1[]"
  Sw_DataStream_1[0Stim|1Ext]/1 -> Bus Creator1/1, Rounding Function/1  "Sw_DataStream_1[0Stim|1Ext]"

== system ASM_Traffic_A11/Environment/Road/UserInterface/PAR_Plant/Objects_DataStreams/DataStream_2 ==
  Maneuver_Signals[] : Inport
  Bus Creator1 : BusCreator  Inputs=4
  Bus Selector : BusSelector  OutputSignals=ManeuverState[]
  Compare To Constant : simulink/Logic and Bit Operations/Compare To Constant  relop=>=  const=3.0  OutDataTypeStr=boolean
  Multiport Switch : MultiPortSwitch  DataPortOrder=Zero-based contiguous  Inputs=2  zeroidx=on  SaturateOnIntegerOverflow=off  InputSameDT=off
  Rounding Function : Rounding  Operator=round
  Saturation : Saturate  UpperLimit=1  LowerLimit=0
  Selector : Selector  InputPortWidth=4  IndexOptions=Index vector (port)  Indices=[1 3]  OutputSizes=1
  Stim_DataStream_2[] : Constant  Value=3
  Sw_DataStream_2[0Stim|1Ext] : Constant
  TrafficLight2_Control : Subsystem
  TrafficLightState[1Red|2Yellow|3RedYellow|4Green] : Constant  Value=[1 3 4 2]  VectorParams1D=off
  DataStream_2[] : Outport  VectorParamsAs1DForOutWhenUnconnected=off
  wires:
  Sw_DataStream_2[0Stim|1Ext]/1 -> Rounding Function/1, Bus Creator1/1  "Sw_DataStream_2[0Stim|1Ext]"
  TrafficLight2_Control/1(TrafficLightState[1|2|3|4]) -> Bus Creator1/3, Multiport Switch/3  "Ext_DataStream_2[]"
  Rounding Function/1 -> Saturation/1
  Saturation/1 -> Multiport Switch/1
  Multiport Switch/1 -> Bus Creator1/4  "DataStream_2[]"
  Selector/1 -> Multiport Switch/2, Bus Creator1/2  "Stim_DataStream_2[]"
  Bus Creator1/1 -> DataStream_2[]/1
  Stim_DataStream_2[]/1 -> Selector/2
  Maneuver_Signals[]/1 -> Bus Selector/1
  Bus Selector/1 -> Compare To Constant/1  "<ManeuverState[]>"
  Compare To Constant/1 -> TrafficLight2_Control/1(Reset[])
  TrafficLightState[1Red|2Yellow|3RedYellow|4Green]/1 -> Selector/1

== system ASM_Traffic_A11/Environment/Road/UserInterface/PAR_Plant/Objects_DataStreams/DataStream_3 ==
  Maneuver_Signals[] : Inport
  Bus Creator1 : BusCreator  Inputs=4
  Bus Selector : BusSelector  OutputSignals=ManeuverState[]
  Compare To Constant : simulink/Logic and Bit Operations/Compare To Constant  relop=>=  const=3.0  OutDataTypeStr=boolean
  Multiport Switch : MultiPortSwitch  DataPortOrder=Zero-based contiguous  Inputs=2  zeroidx=on  SaturateOnIntegerOverflow=off  InputSameDT=off
  Rounding Function : Rounding  Operator=round
  Saturation : Saturate  UpperLimit=1  LowerLimit=0
  Selector : Selector  InputPortWidth=4  IndexOptions=Index vector (port)  Indices=[1 3]  OutputSizes=1
  Stim_DataStream_3[] : Constant  Value=3
  Sw_DataStream_3[0Stim|1Ext] : Constant
  TrafficLight3_Control : Subsystem
  TrafficLightState[1Red|2Yellow|3RedYellow|4Green] : Constant  Value=[1 3 4 2]  VectorParams1D=off
  DataStream_3[] : Outport  VectorParamsAs1DForOutWhenUnconnected=off
  wires:
  Compare To Constant/1 -> TrafficLight3_Control/1(Reset[])
  Bus Selector/1 -> Compare To Constant/1  "<ManeuverState[]>"
  Maneuver_Signals[]/1 -> Bus Selector/1
  Stim_DataStream_3[]/1 -> Selector/2
  Bus Creator1/1 -> DataStream_3[]/1
  Selector/1 -> Bus Creator1/2, Multiport Switch/2  "Stim_DataStream_3[]"
  Multiport Switch/1 -> Bus Creator1/4  "DataStream_3[]"
  Saturation/1 -> Multiport Switch/1
  Rounding Function/1 -> Saturation/1
  TrafficLight3_Control/1(TrafficLightState[1|2|3|4]) -> Multiport Switch/3, Bus Creator1/3  "Ext_DataStream_3[]"
  Sw_DataStream_3[0Stim|1Ext]/1 -> Bus Creator1/1, Rounding Function/1  "Sw_DataStream_3[0Stim|1Ext]"
  TrafficLightState[1Red|2Yellow|3RedYellow|4Green]/1 -> Selector/1

== system ASM_Traffic_A11/Environment/Road/UserInterface/PAR_Plant/Objects_DataStreams/DataStream_4 ==
  Maneuver_Signals[] : Inport
  Bus Creator1 : BusCreator  Inputs=4
  Bus Selector : BusSelector  OutputSignals=ManeuverState[]
  Compare To Constant : simulink/Logic and Bit Operations/Compare To Constant  relop=>=  const=3.0  OutDataTypeStr=boolean
  Multiport Switch : MultiPortSwitch  DataPortOrder=Zero-based contiguous  Inputs=2  zeroidx=on  SaturateOnIntegerOverflow=off  InputSameDT=off
  Rounding Function : Rounding  Operator=round
  Saturation : Saturate  UpperLimit=1  LowerLimit=0
  Selector2 : Selector  InputPortWidth=4  IndexOptions=Index vector (port)  Indices=[1 3]  OutputSizes=1
  Stim_DataStream_4[] : Constant  Value=3
  Sw_DataStream_4[0Stim|1Ext] : Constant
  TrafficLight4_Control : Subsystem
  TrafficLightState[1Red|2Yellow|3RedYellow|4Green] : Constant  Value=[1 3 4 2]  VectorParams1D=off
  DataStream_4[] : Outport  VectorParamsAs1DForOutWhenUnconnected=off
  wires:
  Sw_DataStream_4[0Stim|1Ext]/1 -> Rounding Function/1, Bus Creator1/1  "Sw_DataStream_4[0Stim|1Ext]"
  TrafficLight4_Control/1(TrafficLightState[1|2|3|4]) -> Bus Creator1/3, Multiport Switch/3  "Ext_DataStream_4[]"
  Rounding Function/1 -> Saturation/1
  Saturation/1 -> Multiport Switch/1
  Multiport Switch/1 -> Bus Creator1/4  "DataStream_4[]"
  Selector2/1 -> Multiport Switch/2, Bus Creator1/2  "Stim_DataStream_4[]"
  Bus Creator1/1 -> DataStream_4[]/1
  Stim_DataStream_4[]/1 -> Selector2/2
  TrafficLightState[1Red|2Yellow|3RedYellow|4Green]/1 -> Selector2/1
  Maneuver_Signals[]/1 -> Bus Selector/1
  Bus Selector/1 -> Compare To Constant/1  "<ManeuverState[]>"
  Compare To Constant/1 -> TrafficLight4_Control/1(Reset[])
